simulink model "hrg_wa_v9_identification"  (R2025a)
settings: Solver=ode4  StartTime=0.0  StopTime=20  FixedStep=0.0050000000000000001  RelTol=1e-3
settings Model: Creator=11725  LastModifiedBy=11725

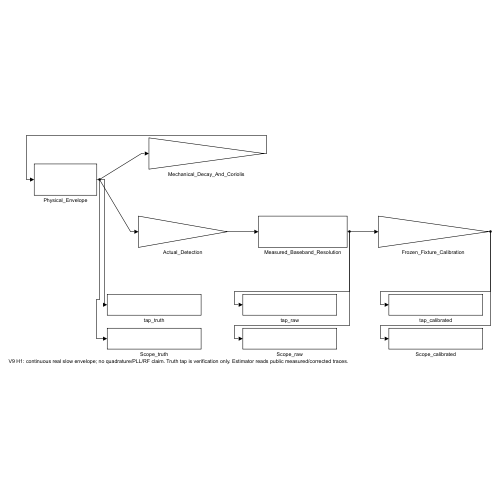
[thumbnail: Simulink's stored preview of the top-level diagram]
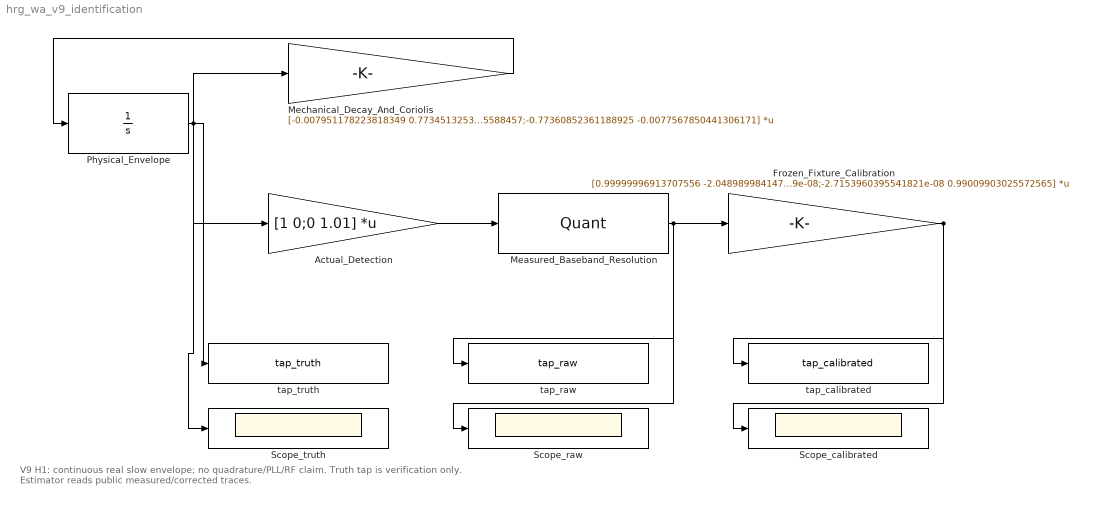
== system hrg_wa_v9_identification ==
  note: V9 H1: continuous real slow envelope; no quadrature/PLL/RF claim. Truth tap is verification only. Estimator reads public measured/corrected traces.
  Actual_Detection : Gain  Gain=[1 0;0 1.01]  Multiplication=Matrix(K*u)
  Frozen_Fixture_Calibration : Gain  Gain=[0.99999996913707556 -2.0489899841476379e-08;-2.7153960395541821e-08 0.99009903025572565]  Multiplication=Matrix(K*u)
  Measured_Baseband_Resolution : Quantizer  QuantizationInterval=9.5367431640625e-07
  Mechanical_Decay_And_Coriolis : Gain  Gain=[-0.007951178223818349 0.77345132535588457;-0.77360852361188925 -0.0077567850441306171]  Multiplication=Matrix(K*u)
  Physical_Envelope : Integrator  InitialCondition=[0.96269626330737756;0.27058437614543168]
  Scope_calibrated : Scope
  Scope_raw : Scope
  Scope_truth : Scope
  tap_calibrated : ToWorkspace  VariableName=tap_calibrated  SaveFormat=Timeseries  SampleTime=-1
  tap_raw : ToWorkspace  VariableName=tap_raw  SaveFormat=Timeseries  SampleTime=-1
  tap_truth : ToWorkspace  VariableName=tap_truth  SaveFormat=Timeseries  SampleTime=-1
  wires:
  Physical_Envelope/1 -> Mechanical_Decay_And_Coriolis/1, Actual_Detection/1, tap_truth/1, Scope_truth/1
  Mechanical_Decay_And_Coriolis/1 -> Physical_Envelope/1
  Actual_Detection/1 -> Measured_Baseband_Resolution/1
  Measured_Baseband_Resolution/1 -> Frozen_Fixture_Calibration/1, tap_raw/1, Scope_raw/1
  Frozen_Fixture_Calibration/1 -> tap_calibrated/1, Scope_calibrated/1
